simulink model "LabA_LinearizedBotVsSimulator"  (R2025b)
settings: Solver=ode14x  StartTime=0.0  StopTime=5  FixedStep=0.001  RelTol=1e-2  EnableMultiTasking=on
undefined symbols (not defined in the file or in its folder): A, B, C, D, Kd, Ki, Kp, sigbuilder_block
libraries: slpidlib x2, cstblocks x1
Description:
  | Real-Time Van der Pol Simulation
  | 
  | This model shows a real-time version of the Simulink(R) Van der Pol
  | simulation model. This model does not need any external signals, so it does
  | not need any data acquisition hardware or driver. This makes the model ideal
  | for first experiments with Simulink Desktop Real-Time(TM), without need to
  | worry about proper I/O hardware configuration.
  | 
  | How to run this model in Normal Mode:
  | 
  | 1) Double-click the orange button to switch to Normal Mode if needed.
  | 2) Start the real-time execution using Simulation->Run.
  | 3) Observe any missed ticks on the Missed Ticks scope.
  | 
  | How to run this model in External Mode:
  | 
  | 1) Double-click the orange button to switch to External Mode if needed.
  | 2) Start the real-time execution using Simulation->Run. The model will automatically
  |    build, connect to Simulink in External Mode and start.
  | 3) Missed ticks will be always zero.
settings Model: ExtModeTrigDuration=101  Creator=The MathWorks Inc.  LastModifiedBy=lizar
settings SolverCC: AlgebraicLoopSolver=TrustRegion
settings DataIOCC: LimitDataPoints=on  SaveFormat=Array  ReturnWorkspaceOutputs=off  SignalLoggingName=logsOut
settings OptimizationCC: ExpressionDepthLimit=2147483647.0  InitFltsAndDblsToZero=on  EfficientMapNaN2IntZero=off
settings DebuggingCC: UnderspecifiedInitializationDetection=Classic  MergeDetectMultiDrivingBlocksExec=none  SignalResolutionControl=TryResolveAllWithWarning  FcnCallInpInsideContextMsg=warning  UnconnectedInputMsg=warning  UnconnectedOutputMsg=warning  UnconnectedLineMsg=warning  StateNameClashWarn=warning  SFUnexpectedBacktrackingDiag=warning  SFNoUnconditionalDefaultTransitionDiag=warning  SFExecutionAtInitializationDiag=none  ArithmeticOperatorsInVariantConditions=warning
settings HardwareCC: ProdBitPerLong=64.0  ProdHWDeviceType=Intel->x86-64 (Linux 64)  TargetBitPerLong=64.0  TargetBitPerPointer=64.0  TargetIntDivRoundTo=Zero  TargetEndianess=LittleEndian  TargetWordSize=64.0  TargetHWDeviceType=Intel->x86-64
settings ModelReferenceCC: EnableRefExpFcnMdlSchedulingChecks=on  PropagateSignalLabelsOutOfModel=off
settings SFSimCC: SimUseLocalCustomCode=off  CustomCodeUndefinedFunction=UseInterfaceOnly
settings RTWCC: SystemTargetFile=sldrt.tlc  TemplateMakefile=sldrt.tmf  RTWUseLocalCustomCode=off  RTWCompilerOptimization=on  GPUComputeCapability=3.5  Description=Simulink Desktop Real-Time
settings CodeAppCC: MaxIdLength=95.0  StateflowObjectComments=on
settings SimulinkDesktopRealTimeCC: ExtModeTransport=0.0  ExtModeStaticAllocSize=1000000.0  TargetLibSuffix=_sldrt.a  TargetPreCompLibLocation=C:\Program Files\MATLAB\R2025b\toolbox\sldrt\lib\win64  TargetLangStandard=C89/C90 (ANSI)  MultiwordLength=2048.0  DynamicStringBufferSize=256.0  ParMdlRefBuildCompliant=on  PreserveMATLABNamespacesInGeneratedCode=on  SubcomponentCodeInterfacePackaging=Reusable function  SupportVariableSizeSignals=off
settings ConfigComp: CovMetricSettings=dw  CovSaveCumulativeToWorkspaceVar=on  CovSaveSingleToWorkspaceVar=on  CovExternalEMLEnable=off  CovSFcnEnable=off

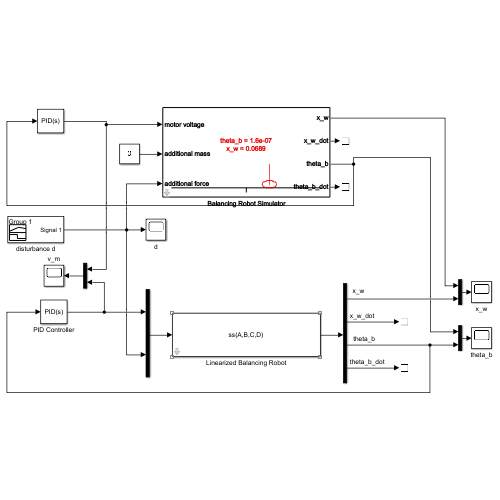
[thumbnail: Simulink's stored preview of the top-level diagram]
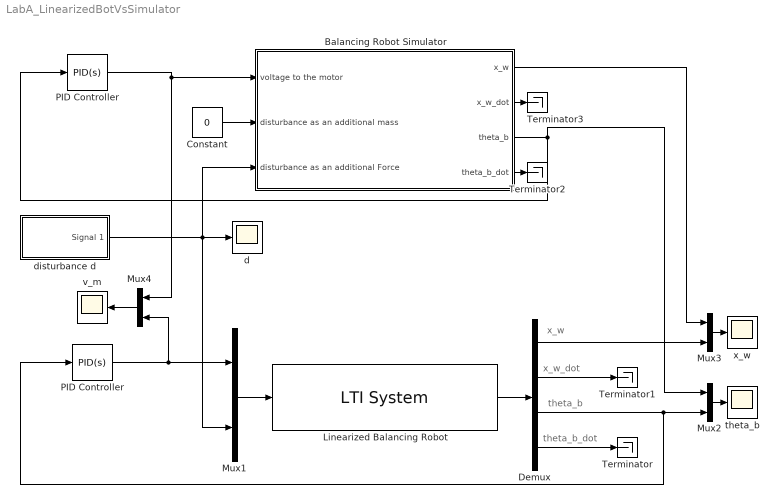
== system LabA_LinearizedBotVsSimulator ==
  note: x_w_dot
  note: x_w
  note: theta_b
  note: theta_b_dot
  Balancing Robot Simulator : Subsystem  mask(Balancing Robot Simulator Parameters){g=9.8, m_b=0.381, l_b=0.112, I_b=0.00616, m_w=0.036, l_w=0.021, I_w=0.00000746, R_m=4.4, L_m=0, b_m=0, b_f=0, K_e=0.444, K_t=0.470, X_0=0, x_w=0.068898, Theta=2.7919e-09, circle_x=0, circle_y=0, scale=2, v_m_limit=9, Theta_0=0*pi/180, x_w_0=0, sigma2_angle=0}
      mask prompts: g "gravitational acceleration"; m_b "mass of the body [kg]"; l_b "length of the body [m]"; I_b "moment of inertia of the body [kg m^2]"; m_w "mass of the wheels [kg]"; l_w "radius of the wheels [m]"; I_w "moment of inertia of the wheels [kg m^2]"; R_m "electrical resistance of the motor [Ohm]"; L_m "electrical inductance of the motor [Henry]"; b_m "viscuous coefficient of the motor"; b_f "wheels - ground friction coefficient"; K_e "back EMF constant of the motor"; K_t "torque constant of the motor"; circle_x "Circl_x"; circle_y "Circl_y"; v_m_limit "saturation limits for the motor voltage"; Theta_0 "initial angle of the body"; x_w_0 "initial position of the wheels"; sigma2_angle "variance of the angle measurement noise"
      mask init:
      | hBlk=get_param(gcb,'Handle');
      | 
      | X_0=[Theta_0 0 x_w_0 0];
      | %%% calculate the circle
      | 
      | r=l_w ;
      | x=-r:r/10:r;
      | circle_y=r*[sqrt(1-x.^2/r^2), -sqrt(1-x.^2/r^2) ]+r;
      | circle_x=[x,x([length(x):-1:1])];
      mask DialogControl PhysicalParametersTab Prompt: Physical parameters
      mask DialogControl InitialConditionsTab Prompt: Initial conditions
      mask DialogControl MeasurementsSystemParametersTab Prompt: Measurement system parameters
      mask Display:
      | color('black');
      | plot([0.0,0.0,1 ,1,0 ],[1,0,0,1,1])
      | port_label('input',		1,  'motor voltage')
      | port_label('input',		2,  'additional mass')
      | port_label('input',		3,  'additional force')
      | port_label('output',	1,	'x_w')
      | port_label('output',	2,	'x_w_dot')
      | port_label('output',	3,	'theta_b')
      | port_label('output',	4,	'theta_b_dot')
      | 
      | x_b = x_w + l_b * sin(Theta);
      | y_b = l_w + l_b * cos(Theta);
      | 
      | Y_OFF = 0.1;
      | X_OFF = 0.5;
      | 
      | plot([0.05,0.95],[Y_OFF,Y_OFF])
      | plot([0.5,0.5],[Y_OFF/2,Y_OFF])
      | 
      | color('r');
      | plot(	(circle_x+x_w)*scale +X_OFF,	...
      | 		(circle_y)*scale+Y_OFF			);
      | 
      | plot(	[x_w x_b] * scale + X_OFF,	...
      | 		[l_w y_b] * scale + Y_OFF	);
      | 
      | color('r');
      | text(0.5, 0.5,																	...
      | 	['theta_b = ' num2str(Theta*180/pi,3) char(10) 'x_w = ' num2str(x_w,3)],		...
      | 	'HorizontalAlignment',	'center',											...
      |     'VerticalAlignment',	'bottom'											);
  Constant : Constant  Value=0
  Demux : Demux
  Linearized Balancing Robot : cstblocks/LTI System  sys=ss(A,B,C,D)  IC=[0 0 0*pi/180 0]  PadeOrder=0
  Mux{1..4} (4 alike) : Mux  Inputs=2
  PID Controller : slpidlib/PID Controller  Controller=PID  Form=Parallel  TimeDomain=Continuous-time  UseExternalTs=off  SampleTime=-1  IntegratorMethod=Forward Euler  FilterMethod=Forward Euler  ControllerParametersSource=internal  P=-Kp  I=-Ki  UseKiTs=off  D=-Kd  UseExternalDerivativeSource=off  N=100000  UseFilter=on  TunerSelectOption=Transfer Function Based (PID Tuner App)  InitialConditionSource=internal  InitialConditionForIntegrator=0  InitialConditionForFilter=0  DifferentiatorICPrevScaledInput=0  ExternalReset=none  TrackingMode=off  Kt=1  LimitOutput=off  SatLimitsSource=internal  UpperSaturationLimit=9  LowerSaturationLimit=-9  LinearizeAsGain=on  AntiWindupMode=clamping  Kb=1  LimitIntegrator=off  UpperIntegratorSaturationLimit=inf  LowerIntegratorSaturationLimit=-inf  POutMin=[]  POutMax=[]  IOutMin=[]  IOutMax=[]  DOutMin=[]  DOutMax=[]  NOutMin=[]  NOutMax=[]  SumOutMin=[]  SumOutMax=[]  SaturationOutMin=[]  SaturationOutMax=[]  PParamMin=[]  PParamMax=[]  IParamMin=[]  IParamMax=[]  DParamMin=[]  DParamMax=[]  NParamMin=[]  NParamMax=[]  KbParamMin=[]  KbParamMax=[]  KtParamMin=[]  KtParamMax=[]  KbOutMin=[]  KbOutMax=[]  KtOutMin=[]  KtOutMax=[]  IntegratorOutMin=[]  IntegratorOutMax=[]  FilterOutMin=[]  FilterOutMax=[]  SumI1OutMin=[]  SumI1OutMax=[]  SumI2OutMin=[]  SumI2OutMax=[]  SumI3OutMin=[]  SumI3OutMax=[]  SumI4OutMin=[]  SumI4OutMax=[]  SumDOutMin=[]  SumDOutMax=[]  DifferentiatorOutMin=[]  DifferentiatorOutMax=[]  FilterDiffOutCoefMin=[]  FilterDiffOutCoefMax=[]  ReciprocalOutMin=[]  ReciprocalOutMax=[]  SumDenOutMin=[]  SumDenOutMax=[]  SumNumOutMin=[]  SumNumOutMax=[]  DivideOutMin=[]  DivideOutMax=[]  UdiffTsProdOutMin=[]  UdiffTsProdOutMax=[]  NTsProdOutMin=[]  NTsProdOutMax=[]  UintegralTsProdOutMin=[]  UintegralTsProdOutMax=[]  UngainTsProdOutMin=[]  UngainTsProdOutMax=[]  ClampingZeroOutDataTypeStr=Inherit: Inherit via back propagation  ClampingZeroOutMin=[]  ClampingZeroOutMax=[]  FilterDenConstantOutDataTypeStr=Inherit: Inherit via back propagation  FilterDenConstantOutMin=[]  FilterDenConstantOutMax=[]  PCopyOutDataTypeStr=Inherit: Inherit via back propagation  PCopyOutMin=[]  PCopyOutMax=[]  NCopyOutDataTypeStr=Inherit: Inherit via back propagation  NCopyOutMin=[]  NCopyOutMax=[]  IntegratorContinuousStateAttributes=''  IntegratorStateMustResolveToSignalObject=off  IntegratorRTWStateStorageClass=Auto  FilterContinuousStateAttributes=''  FilterStateMustResolveToSignalObject=off  FilterRTWStateStorageClass=Auto  ParallelPVariant=InternalParameters  IdealPVariant=Disabled  IVariant=InternalParameters  DVariant=InternalParameters  IntegratorVariant=Continuous  SatVariant=Disabled  AWVariant=Passthrough  PCopyVariant=Disabled  TRVariant=Disabled  FdbkBlocksVariant=Forward  IdealPFdbkVariant=Disabled  SatFdbkVariant=Disabled  DerivativeFilterVariant=ContFilter  NVariant=InternalParameters  NCopyVariant=Disabled  FilterICVariant=InternalICsFilter  IntegratorICVariant=InternalICs  ExternalResetVariant=Disabled  TRSumVariant=Passthrough  SumFdbkVariant=Disabled  SumVariant=Sum_PID  TsampFilterVariant=InternalTs  TsampNgainVariant=Passthrough  TsampIntegralVariant=Disabled_SignalSpec  ExternalSaturationOutDataTypeStr=Inherit: Same as second input  DerivativeSourceVariant=ErrorSignal  PreIntVariant=InternalPreInt
  "PID Controller " : slpidlib/PID Controller  Controller=PID  Form=Parallel  TimeDomain=Continuous-time  UseExternalTs=off  SampleTime=-1  IntegratorMethod=Forward Euler  FilterMethod=Forward Euler  ControllerParametersSource=internal  P=-Kp  I=-Ki  UseKiTs=off  D=-Kd  UseExternalDerivativeSource=off  N=100000  UseFilter=on  TunerSelectOption=Transfer Function Based (PID Tuner App)  InitialConditionSource=internal  InitialConditionForIntegrator=0  InitialConditionForFilter=0  DifferentiatorICPrevScaledInput=0  ExternalReset=none  TrackingMode=off  Kt=1  LimitOutput=off  SatLimitsSource=internal  UpperSaturationLimit=inf  LowerSaturationLimit=-inf  LinearizeAsGain=on  AntiWindupMode=none  Kb=1  LimitIntegrator=off  UpperIntegratorSaturationLimit=inf  LowerIntegratorSaturationLimit=-inf  POutMin=[]  POutMax=[]  IOutMin=[]  IOutMax=[]  DOutMin=[]  DOutMax=[]  NOutMin=[]  NOutMax=[]  SumOutMin=[]  SumOutMax=[]  SaturationOutMin=[]  SaturationOutMax=[]  PParamMin=[]  PParamMax=[]  IParamMin=[]  IParamMax=[]  DParamMin=[]  DParamMax=[]  NParamMin=[]  NParamMax=[]  KbParamMin=[]  KbParamMax=[]  KtParamMin=[]  KtParamMax=[]  KbOutMin=[]  KbOutMax=[]  KtOutMin=[]  KtOutMax=[]  IntegratorOutMin=[]  IntegratorOutMax=[]  FilterOutMin=[]  FilterOutMax=[]  SumI1OutMin=[]  SumI1OutMax=[]  SumI2OutMin=[]  SumI2OutMax=[]  SumI3OutMin=[]  SumI3OutMax=[]  SumI4OutMin=[]  SumI4OutMax=[]  SumDOutMin=[]  SumDOutMax=[]  DifferentiatorOutMin=[]  DifferentiatorOutMax=[]  FilterDiffOutCoefMin=[]  FilterDiffOutCoefMax=[]  ReciprocalOutMin=[]  ReciprocalOutMax=[]  SumDenOutMin=[]  SumDenOutMax=[]  SumNumOutMin=[]  SumNumOutMax=[]  DivideOutMin=[]  DivideOutMax=[]  UdiffTsProdOutMin=[]  UdiffTsProdOutMax=[]  NTsProdOutMin=[]  NTsProdOutMax=[]  UintegralTsProdOutMin=[]  UintegralTsProdOutMax=[]  UngainTsProdOutMin=[]  UngainTsProdOutMax=[]  ClampingZeroOutDataTypeStr=Inherit: Inherit via back propagation  ClampingZeroOutMin=[]  ClampingZeroOutMax=[]  FilterDenConstantOutDataTypeStr=Inherit: Inherit via back propagation  FilterDenConstantOutMin=[]  FilterDenConstantOutMax=[]  PCopyOutDataTypeStr=Inherit: Inherit via back propagation  PCopyOutMin=[]  PCopyOutMax=[]  NCopyOutDataTypeStr=Inherit: Inherit via back propagation  NCopyOutMin=[]  NCopyOutMax=[]  IntegratorContinuousStateAttributes=''  IntegratorStateMustResolveToSignalObject=off  IntegratorRTWStateStorageClass=Auto  FilterContinuousStateAttributes=''  FilterStateMustResolveToSignalObject=off  FilterRTWStateStorageClass=Auto  ParallelPVariant=InternalParameters  IdealPVariant=Disabled  IVariant=InternalParameters  DVariant=InternalParameters  IntegratorVariant=Continuous  SatVariant=Disabled  AWVariant=Passthrough  PCopyVariant=Disabled  TRVariant=Disabled  FdbkBlocksVariant=Forward  IdealPFdbkVariant=Disabled  SatFdbkVariant=Disabled  DerivativeFilterVariant=ContFilter  NVariant=InternalParameters  NCopyVariant=Disabled  FilterICVariant=InternalICsFilter  IntegratorICVariant=InternalICs  ExternalResetVariant=Disabled  TRSumVariant=Passthrough  SumFdbkVariant=Disabled  SumVariant=Sum_PID  TsampFilterVariant=InternalTs  TsampNgainVariant=Passthrough  TsampIntegralVariant=Disabled_SignalSpec  ExternalSaturationOutDataTypeStr=Inherit: Same as second input  DerivativeSourceVariant=ErrorSignal  PreIntVariant=InternalPreInt
  Terminator{,1..3} (4 alike) : Terminator
  d : Scope
      settings: DataLoggingVariableName=d
  disturbance d : Subsystem  Tag=STV Subsys  LoadFcn=sigbuilder_block('load');  StartFcn=sigbuilder_block('start');  StopFcn=sigbuilder_block('stop');  ClipboardFcn=sigbuilder_block('clipboard');  mask(Sigbuilder block){tuvar=[0:10]}
      mask help: Simulink:masks:SigbuilderBlock_MD
      mask init:
      | if ~strcmp(get_param(bdroot(gcbh),'SimulationStatus'),'stopped') tuvar = sigbuilder_block('maskInit'); end
      settings: CopyFcn=sigbuilder_block('copy');  DeleteFcn=sigbuilder_block('delete');  ModelCloseFcn=sigbuilder_block('modelClose');  PreSaveFcn=sigbuilder_block('preSave');  PauseFcn=sigbuilder_block('pause');  ContinueFcn=sigbuilder_block('continue');  NameChangeFcn=sigbuilder_block('namechange');  OpenFcn=sigbuilder_block('open',[437.6 199.2 550.4 400 ]);  CloseFcn=sigbuilder_block('close');
      mask Display: plot(0, 0, 100, 100,[2, 2, 32, 32, 2], [68, 8, 8, 68, 68],[32, 2], [38, 38], [32, 19, 2],[53, 60, 44], [32, 17, 17, 2],[16, 16, 31, 31]);txt = getActiveGroup(gcbh);text(2, 100, txt,'verticalAlignment', 'top');
  theta_b : Scope
      settings: ActiveDisplayYMinimum=-0.00022064222182481929  ActiveDisplayYMaximum=0.0019857799964233739  DataLoggingVariableName=theta_b
  v_m : Scope
      settings: ActiveDisplayYMinimum=-1  ActiveDisplayYMaximum=1  DataLoggingVariableName=v_m
  x_w : Scope
      settings: ActiveDisplayYMinimum=-0.0086122620040747586  ActiveDisplayYMaximum=0.077510358036672847  DataLoggingVariableName=x_w
  wires:
  PID Controller/1 -> Mux4/1, Balancing Robot Simulator/1(voltage to the motor)
  Mux1/1 -> Linearized Balancing Robot/1
  Linearized Balancing Robot/1 -> Demux/1
  disturbance d/1(Signal 1) -> Mux1/2, Balancing Robot Simulator/3(disturbance as an additional Force), d/1
  Balancing Robot Simulator/3(theta_b) -> Mux2/1, PID Controller/1
  Balancing Robot Simulator/1(x_w) -> Mux3/1
  Mux3/1 -> x_w/1
  Mux2/1 -> theta_b/1
  Demux/1 -> Mux3/2
  Demux/3 -> Mux2/2, "PID Controller "/1
  "PID Controller "/1 -> Mux4/2, Mux1/1
  Mux4/1 -> v_m/1
  Demux/2 -> Terminator1/1
  Demux/4 -> Terminator/1
  Balancing Robot Simulator/4("theta_b_dot ") -> Terminator2/1
  Balancing Robot Simulator/2(x_w_dot) -> Terminator3/1
  Constant/1 -> Balancing Robot Simulator/2("disturbance as an additional mass ")

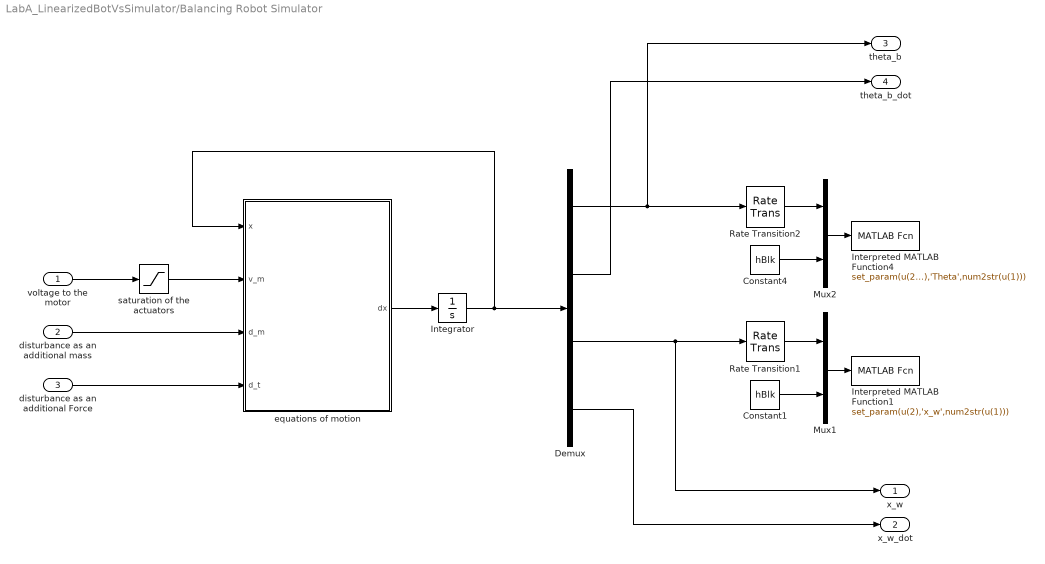
== system LabA_LinearizedBotVsSimulator/Balancing Robot Simulator ==
  voltage to the motor : Inport
  "disturbance as an additional mass " : Inport  Port=2
  disturbance as an additional Force : Inport  Port=3
  Constant1 : Constant  Value=hBlk
  Constant4 : Constant  Value=hBlk
  Demux : Demux
  Integrator : Integrator  InitialCondition=X_0
  Interpreted MATLAB Function1 : MATLABFcn  MATLABFcn=set_param(u(2),'x_w',num2str(u(1)))  OutputDimensions=0  SampleTime=0.1
  Interpreted MATLAB Function4 : MATLABFcn  MATLABFcn=set_param(u(2),'Theta',num2str(u(1)))  OutputDimensions=0
  Mux1 : Mux  Inputs=2
  Mux2 : Mux  Inputs=2
  Rate Transition1 : RateTransition  OutPortSampleTime=0.1
  Rate Transition2 : RateTransition  OutPortSampleTime=0.1
  equations of motion : MATLAB Function  TreatAsAtomicUnit=on
  saturation of the actuators : Saturate  UpperLimit=v_m_limit  LowerLimit=-v_m_limit
  x_w : Outport
  x_w_dot : Outport  Port=2
  theta_b : Outport  Port=3
  "theta_b_dot " : Outport  Port=4
  wires:
  Integrator/1 -> equations of motion/1(x), Demux/1
  Constant4/1 -> Mux2/2
  Mux2/1 -> Interpreted MATLAB Function4/1
  Rate Transition2/1 -> Mux2/1
  equations of motion/1(dx) -> Integrator/1
  voltage to the motor/1 -> saturation of the actuators/1
  Constant1/1 -> Mux1/2
  Mux1/1 -> Interpreted MATLAB Function1/1
  Rate Transition1/1 -> Mux1/1
  Demux/3 -> x_w/1, Rate Transition1/1
  saturation of the actuators/1 -> equations of motion/2(v_m)
  "disturbance as an additional mass "/1 -> equations of motion/3(d_m)
  disturbance as an additional Force/1 -> equations of motion/4(d_t)
  Demux/1 -> theta_b/1, Rate Transition2/1
  Demux/2 -> "theta_b_dot "/1
  Demux/4 -> x_w_dot/1

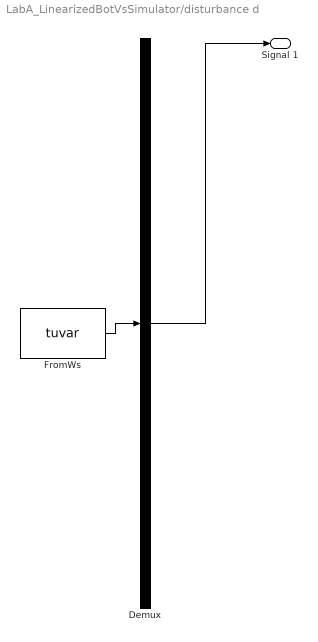
== system LabA_LinearizedBotVsSimulator/disturbance d ==
  Demux : Demux  Tag=STV Demux  Outputs=1
      settings: DisplayOption=none
  FromWs : FromWorkspace  Tag=STV FromWs  VariableName=tuvar
      SigBuilderData=|
      | common.afterFinalStr = 'Extrapolate'
      | common.sampleTime = 0
      | dataSet.timeRange = [0 10]
      | dataSet.name = 'Group 1'
      | sbobj.Groups.Name = 'Group 1'
      | sbobj.Groups.Signals.Name = 'Signal 1'
      | sbobj.Groups.Signals.XData = [0 0.1 0.1 10]
      | sbobj.Groups.Signals.YData = [0.02 0.02 0 0]
  Signal 1 : Outport  Tag=STV Outport
  wires:
  Demux/1 -> Signal 1/1
  FromWs/1 -> Demux/1

== matlab function LabA_LinearizedBotVsSimulator/Balancing Robot Simulator/equations of motion ==
  data: x input; dx output; v_m input; d_m input; d_t input; g parameter; b_f parameter; m_b parameter; l_b parameter; I_b parameter; m_w parameter; l_w parameter; I_w parameter; R_m parameter; L_m parameter; b_m parameter; K_e parameter; K_t parameter
function dx = EquationsOfMotion(x,		...
								v_m,	...
								d_m,	... % additional mass on the body
								d_t,	... % Fource that acted on the body
								g,		...
								b_f,	...
								m_b,	...
								l_b,	...
								I_b,	...
								m_w,	...
								l_w,	...
								I_w,	...
								R_m,	...
								L_m,	...
								b_m,	...
								K_e,	...
								K_t		) %#ok<*INUSL>

% initialization of the state
dx = zeros(4,1);

% TODO: the motor electrical inductance and the motor viscous coefficients
% are neglected

% for readability -- state of the system
theta		= x(1);
theta_dot	= x(2);
x_b			= x(3);
x_b_dot		= x(4);

% add the mass disturbance: notice that we need to modify also the
% moment of inertia
m_t_b = m_b + d_m;
I_t_b = I_b * m_t_b / m_b;

% equations of motion (obfuscated)
dx(1)=theta_dot;
dx(2)=((b_f + (K_e*K_t)/R_m)*(theta_dot - x_b_dot/l_w) + (K_t*v_m)/R_m - d_t*l_b*1*cos(theta) - g*l_b*m_t_b*sin(theta) + (l_b*m_t_b*cos(theta)*(d_t*l_w + (b_f + (K_e*K_t)/R_m)*(theta_dot - x_b_dot/l_w) + (K_t*v_m)/R_m + l_b*l_w*m_t_b*theta_dot^2*sin(theta)))/(l_w*m_t_b + l_w*m_w + I_w/l_w))/((m_t_b*l_b^2 + I_t_b)*((l_b^2*l_w*m_t_b^2*cos(theta)^2)/((m_t_b*l_b^2 + I_t_b)*(l_w*m_t_b + l_w*m_w + I_w/l_w)) - 1));
dx(3)=x_b_dot;
dx(4)= -(d_t*l_w + (b_f + (K_e*K_t)/R_m)*(theta_dot - x_b_dot/l_w) + (K_t*v_m)/R_m + l_b*l_w*m_t_b*theta_dot^2*sin(theta) + (l_b*l_w*m_t_b*cos(theta)*((b_f + (K_e*K_t)/R_m)*(theta_dot - x_b_dot/l_w) + (K_t*v_m)/R_m - d_t*l_b*1*cos(theta) - g*l_b*m_t_b*sin(theta)))/(m_t_b*l_b^2 + I_t_b))/(((l_b^2*l_w*m_t_b^2*cos(theta)^2)/((m_t_b*l_b^2 + I_t_b)*(l_w*m_t_b + l_w*m_w + I_w/l_w)) - 1)*(l_w*m_t_b + l_w*m_w + I_w/l_w));

% if the robot falls
if( (x(1) > pi/2) || (x(1) < -pi/2) )
	%
	dx(1) = 0;
	dx(2) = 0;
	dx(3) = 0;
	dx(4) = 0;
	%
end;%


% g   = 9.8;
% b_f = 0;
% m_t_b = 0.381;
% l_b = 0.112;
% I_t_b = 0.00616;
% m_w = 0.036;
% l_w = 0.021;
% I_w = 0.00000746;
% R_m = 4.4;
% L_m = 0 ;
% b_m = 0;
% K_e = 0.444;
% K_t = 0.470;
